simulink model "v1_weekly"  (R2024a)
settings: Solver=ode45  StartTime=0.0  StopTime=6  MaxStep=0.01  RelTol=1e-8  AbsTol=1e-10
model workspace (MAT data in the model file):
  U = 0.4
  m = 2
  t_step = 1
  v0 = 0
  z0 = 0
settings Model: Creator=admin  LastModifiedBy=admin

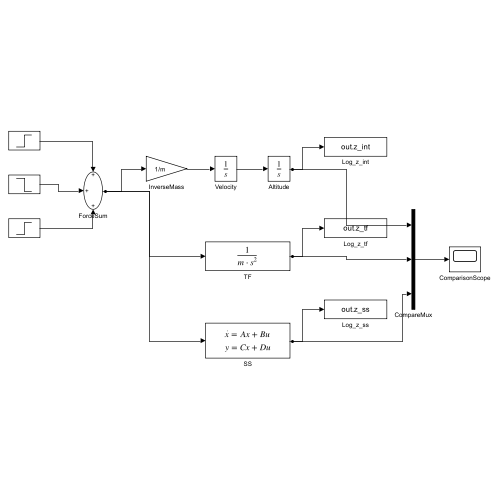
[thumbnail: Simulink's stored preview of the top-level diagram]
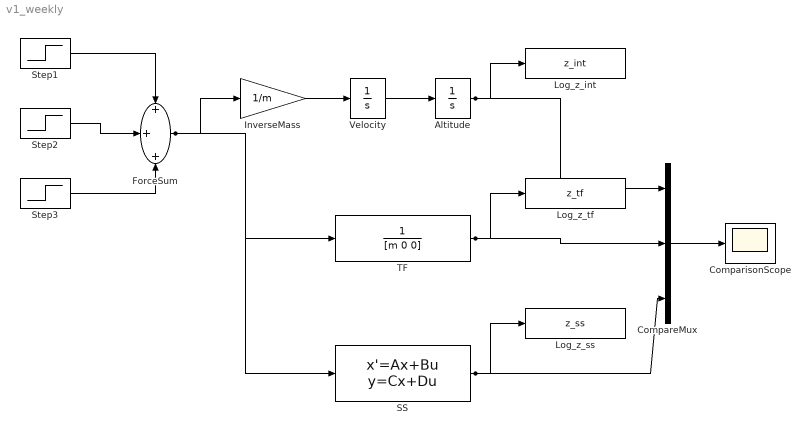
== system v1_weekly ==
  Altitude : Integrator  InitialCondition=z0
  CompareMux : Mux  Inputs=3
  ComparisonScope : Scope
  ForceSum : Sum  Inputs=+++
  InverseMass : Gain  Gain=1/m
  Log_z_int : ToWorkspace  VariableName=z_int  SaveFormat=Timeseries  SampleTime=-1
  Log_z_ss : ToWorkspace  VariableName=z_ss  SaveFormat=Timeseries  SampleTime=-1
  Log_z_tf : ToWorkspace  VariableName=z_tf  SaveFormat=Timeseries  SampleTime=-1
  SS : StateSpace  A=[0 1;0 0]  B=[0;1/m]  C=[1 0]  D=0  InitialCondition=[z0;v0]
  Step1 : Step  After=U  SampleTime=0
  Step2 : Step  Time=3  After=-2*U  SampleTime=0
  Step3 : Step  Time=5  After=U  SampleTime=0
  TF : TransferFcn  Numerator=1  Denominator=[m 0 0]
  Velocity : Integrator  InitialCondition=v0
  wires:
  Step1/1 -> ForceSum/1
  Step2/1 -> ForceSum/2
  Step3/1 -> ForceSum/3
  ForceSum/1 -> InverseMass/1, TF/1, SS/1
  InverseMass/1 -> Velocity/1
  Velocity/1 -> Altitude/1
  CompareMux/1 -> ComparisonScope/1
  Altitude/1 -> Log_z_int/1, CompareMux/1
  TF/1 -> Log_z_tf/1, CompareMux/2
  SS/1 -> Log_z_ss/1, CompareMux/3
